simulink model "BoP_Test_SIL"  (R2026a)
settings: Solver=FixedStepDiscrete  StopTime=9  FixedStep=Ts_ctrl
InitFcn:
  | init_Controller_BoP
undefined symbols (not defined in the file or in its folder): Ts_ctrl
Description:
  | Banco SIL Ball on Plate: ramas Normal y SIL de Controller_BoP (ejes X e Y), cada una con su planta (planta_bop_paso). Ensayo D4.
settings Model: Creator=ablopez@estudiantes.ie.tec.ac.cr  LastModifiedBy=ablopez@estudiantes.ie.tec.ac.cr

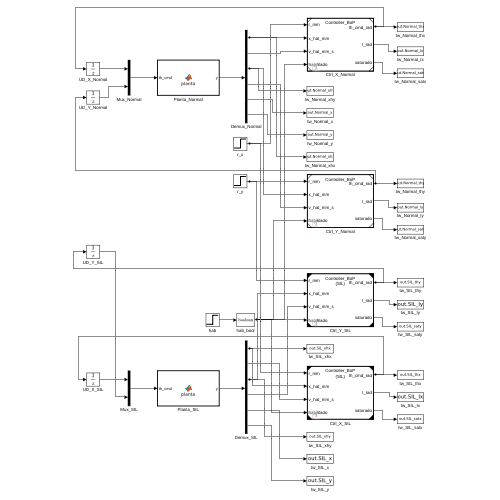
[thumbnail: Simulink's stored preview of the top-level diagram]
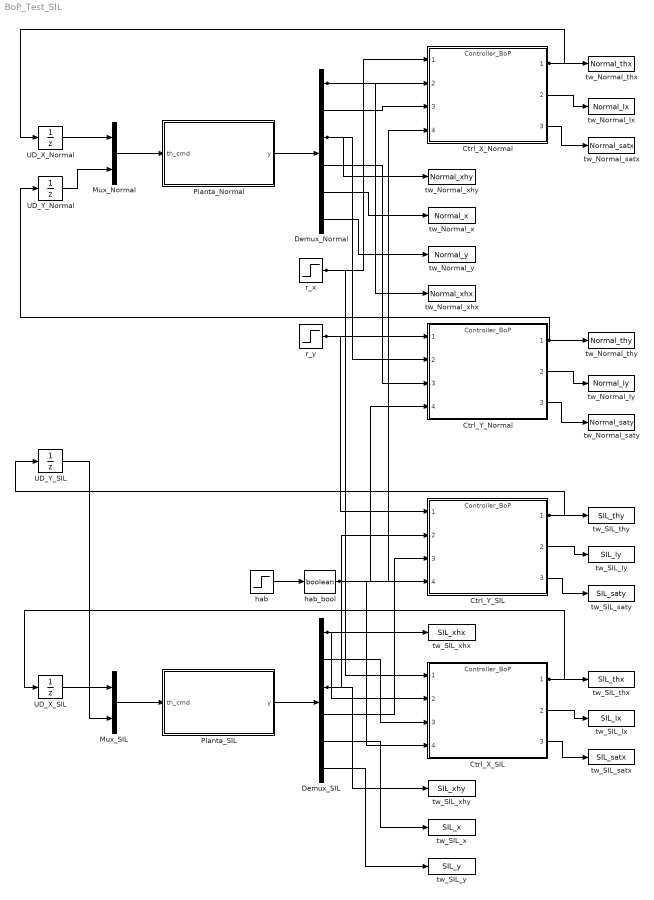
== system BoP_Test_SIL ==
  Ctrl_X_Normal : ModelReference  ModelNameDialog=Controller_BoP  SimulationMode=Normal  ModelReferenceVersion=1.1
  Ctrl_X_SIL : ModelReference  ModelNameDialog=Controller_BoP  SimulationMode=Software-in-the-loop (SIL)  ModelReferenceVersion=1.1
  Ctrl_Y_Normal : ModelReference  ModelNameDialog=Controller_BoP  SimulationMode=Normal  ModelReferenceVersion=1.1
  Ctrl_Y_SIL : ModelReference  ModelNameDialog=Controller_BoP  SimulationMode=Software-in-the-loop (SIL)  ModelReferenceVersion=1.1
  Demux_Normal : Demux  Outputs=6
  Demux_SIL : Demux  Outputs=6
  Mux_Normal : Mux  Inputs=2
  Mux_SIL : Mux  Inputs=2
  Planta_Normal : MATLAB Function  TreatAsAtomicUnit=on
  Planta_SIL : MATLAB Function  TreatAsAtomicUnit=on
  UD_X_Normal : UnitDelay  SampleTime=Ts_ctrl
  UD_X_SIL : UnitDelay  SampleTime=Ts_ctrl
  UD_Y_Normal : UnitDelay  SampleTime=Ts_ctrl
  UD_Y_SIL : UnitDelay  SampleTime=Ts_ctrl
  hab : Step  Time=0.5  SampleTime=Ts_ctrl
  hab_bool : DataTypeConversion  OutDataTypeStr=boolean  SaturateOnIntegerOverflow=off  RndMeth=Floor
  r_x : Step  Time=4.5  FinalValue=50  SampleTime=Ts_ctrl
  r_y : Step  Time=4.5  FinalValue=50  SampleTime=Ts_ctrl
  tw_Normal_Ix : ToWorkspace  VariableName=Normal_Ix  SaveFormat=Timeseries  SampleTime=-1
  tw_Normal_Iy : ToWorkspace  VariableName=Normal_Iy  SaveFormat=Timeseries  SampleTime=-1
  tw_Normal_satx : ToWorkspace  VariableName=Normal_satx  SaveFormat=Timeseries  SampleTime=-1
  tw_Normal_saty : ToWorkspace  VariableName=Normal_saty  SaveFormat=Timeseries  SampleTime=-1
  tw_Normal_thx : ToWorkspace  VariableName=Normal_thx  SaveFormat=Timeseries  SampleTime=-1
  tw_Normal_thy : ToWorkspace  VariableName=Normal_thy  SaveFormat=Timeseries  SampleTime=-1
  tw_Normal_x : ToWorkspace  VariableName=Normal_x  SaveFormat=Timeseries  SampleTime=-1
  tw_Normal_xhx : ToWorkspace  VariableName=Normal_xhx  SaveFormat=Timeseries  SampleTime=-1
  tw_Normal_xhy : ToWorkspace  VariableName=Normal_xhy  SaveFormat=Timeseries  SampleTime=-1
  tw_Normal_y : ToWorkspace  VariableName=Normal_y  SaveFormat=Timeseries  SampleTime=-1
  tw_SIL_Ix : ToWorkspace  VariableName=SIL_Ix  SaveFormat=Timeseries  SampleTime=-1
  tw_SIL_Iy : ToWorkspace  VariableName=SIL_Iy  SaveFormat=Timeseries  SampleTime=-1
  tw_SIL_satx : ToWorkspace  VariableName=SIL_satx  SaveFormat=Timeseries  SampleTime=-1
  tw_SIL_saty : ToWorkspace  VariableName=SIL_saty  SaveFormat=Timeseries  SampleTime=-1
  tw_SIL_thx : ToWorkspace  VariableName=SIL_thx  SaveFormat=Timeseries  SampleTime=-1
  tw_SIL_thy : ToWorkspace  VariableName=SIL_thy  SaveFormat=Timeseries  SampleTime=-1
  tw_SIL_x : ToWorkspace  VariableName=SIL_x  SaveFormat=Timeseries  SampleTime=-1
  tw_SIL_xhx : ToWorkspace  VariableName=SIL_xhx  SaveFormat=Timeseries  SampleTime=-1
  tw_SIL_xhy : ToWorkspace  VariableName=SIL_xhy  SaveFormat=Timeseries  SampleTime=-1
  tw_SIL_y : ToWorkspace  VariableName=SIL_y  SaveFormat=Timeseries  SampleTime=-1
  wires:
  Ctrl_X_SIL/3 -> tw_SIL_satx/1
  Ctrl_X_SIL/1 -> tw_SIL_thx/1, UD_X_SIL/1
  Ctrl_Y_SIL/2 -> tw_SIL_Iy/1
  Ctrl_Y_Normal/3 -> tw_Normal_saty/1
  Demux_Normal/4 -> Ctrl_Y_Normal/3
  Ctrl_X_Normal/2 -> tw_Normal_Ix/1
  Ctrl_Y_Normal/2 -> tw_Normal_Iy/1
  Demux_Normal/2 -> Ctrl_X_Normal/3
  Demux_Normal/1 -> tw_Normal_xhx/1, Ctrl_X_Normal/2
  Ctrl_X_Normal/1 -> tw_Normal_thx/1, UD_X_Normal/1
  Demux_Normal/3 -> tw_Normal_xhy/1, Ctrl_Y_Normal/2
  Ctrl_X_SIL/2 -> tw_SIL_Ix/1
  hab_bool/1 -> Ctrl_Y_SIL/4, Ctrl_X_SIL/4, Ctrl_Y_Normal/4, Ctrl_X_Normal/4
  Planta_SIL/1(y) -> Demux_SIL/1
  Planta_Normal/1(y) -> Demux_Normal/1
  Mux_SIL/1 -> Planta_SIL/1(th_cmd)
  UD_Y_SIL/1 -> Mux_SIL/2
  Mux_Normal/1 -> Planta_Normal/1(th_cmd)
  UD_Y_Normal/1 -> Mux_Normal/2
  Ctrl_Y_SIL/3 -> tw_SIL_saty/1
  Ctrl_Y_SIL/1 -> tw_SIL_thy/1, UD_Y_SIL/1
  UD_X_Normal/1 -> Mux_Normal/1
  Demux_Normal/6 -> tw_Normal_y/1
  Demux_SIL/3 -> tw_SIL_xhy/1, Ctrl_Y_SIL/2
  Demux_Normal/5 -> tw_Normal_x/1
  Demux_SIL/1 -> tw_SIL_xhx/1, Ctrl_X_SIL/2
  r_x/1 -> Ctrl_X_SIL/1, Ctrl_X_Normal/1
  r_y/1 -> Ctrl_Y_SIL/1, Ctrl_Y_Normal/1
  Demux_SIL/2 -> Ctrl_X_SIL/3
  Demux_SIL/4 -> Ctrl_Y_SIL/3
  hab/1 -> hab_bool/1
  Demux_SIL/6 -> tw_SIL_y/1
  Demux_SIL/5 -> tw_SIL_x/1
  Ctrl_X_Normal/3 -> tw_Normal_satx/1
  UD_X_SIL/1 -> Mux_SIL/1
  Ctrl_Y_Normal/1 -> tw_Normal_thy/1, UD_Y_Normal/1

== matlab function BoP_Test_SIL/Planta_Normal ==
  data: th_cmd input; y output
function y = planta(th_cmd)
%#codegen
% Planta del banco: ver etapaF/funciones/planta_bop_paso.m
persistent S
Pp = planta_bop_param();
if isempty(S)
    S = planta_bop_estado0(Pp);
end
[y, S] = planta_bop_paso(th_cmd, S, Pp);
end

== matlab function BoP_Test_SIL/Planta_SIL ==
  data: th_cmd input; y output
function y = planta(th_cmd)
%#codegen
% Planta del banco: ver etapaF/funciones/planta_bop_paso.m
persistent S
Pp = planta_bop_param();
if isempty(S)
    S = planta_bop_estado0(Pp);
end
[y, S] = planta_bop_paso(th_cmd, S, Pp);
end
